simulink model "LQTesting"  (R2025b)
settings: Solver=VariableStepAuto  StartTime=0.0  StopTime=5  RelTol=1e-3
undefined symbols (not defined in the file): ENGINE, IN, K, TANKS, VEH
libraries: simulink_extras x4, aerolibanim x1, matrix_library x1, simulink x1
settings Model: Creator=maxma  LastModifiedBy=maxma

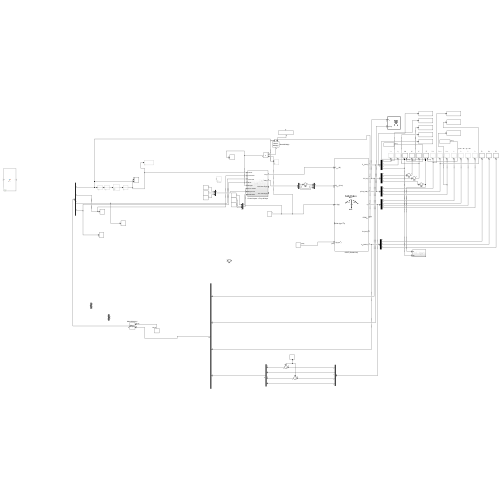
[thumbnail: Simulink's stored preview of the top-level diagram]
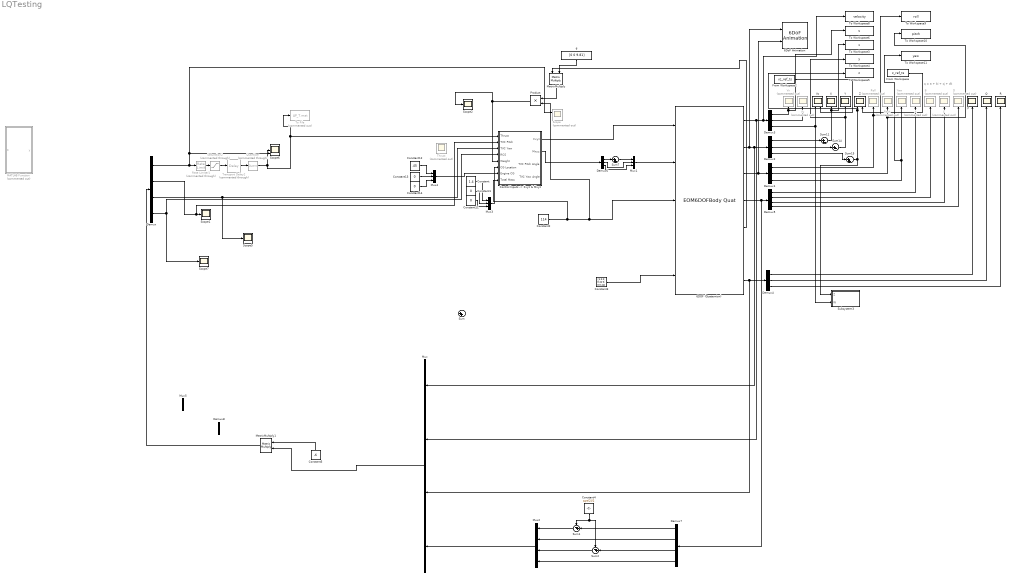
== system LQTesting ==
  note: q = a + bi + cj + dk
  6DOF (Quaternion) : EOM6DOFBodyQuat  mtype=Custom Variable  eul_0=[0 pi/2 0]
  6DoF Animation : aerolibanim/6DoF Animation  u1=[0 200 -200 200 -100 5]  u2=0.1  u3=2  u4=[4000 0 -5000]  u5=Fly alongside  u6=[100 100 -50]  u7=10  u8=on
  A : Scope  Commented=on
      settings: ActiveDisplayYMinimum=-1  ActiveDisplayYMaximum=1  DataLoggingVariableName=ScopeData12
  B : Scope  Commented=on
      settings: ActiveDisplayYMinimum=-1  ActiveDisplayYMaximum=1  DataLoggingVariableName=ScopeData13
  C : Scope  Commented=on
      settings: DataLoggingVariableName=ScopeData14
  Constant : Constant  Value=1.4
  Constant{1,11,13..14} (4 alike) : Constant  Value=0
  Constant12 : Constant  Value=.45
  Constant2 : Constant  Value=114
  Constant3 : Constant  Value=[1 0 0; 0 41 0; 0 0 41]
  Constant4 : Constant  Value=sqrt(2)/2
  Constant5 : Constant  Value=-K
  "Control Inputs -> Fxyz & Mxyz" : Subsystem
  D : Scope  Commented=on
      settings: DataLoggingVariableName=ScopeData15
  Demux{,5,7..8} (4 alike) : Demux
  Demux{1..4,6} (5 alike) : Demux  Outputs=3
  From Workspace : FromWorkspace  VariableName=z_ref_ts
  From Workspace2 : FromWorkspace  VariableName=vz_ref_ts
  MATLAB Function : MATLAB Function  Commented=on  TreatAsAtomicUnit=on
  MatrixMultiply : Product  Multiplication=Matrix(*)
  MatrixMultiply1 : Product  Multiplication=Matrix(*)
  Mux : Mux
  Mux1 : Mux  Inputs=3
  Mux2 : Mux
  Mux3 : Mux  Inputs=3
  Mux4 : Mux  Inputs=3
  Mux5 : Mux  Inputs=2
  P : Scope
      settings: ActiveDisplayYMinimum=-1.1737221275555805  ActiveDisplayYMaximum=1.4340005685452235  DataLoggingVariableName=ScopeData9
  Pitch : Scope  Commented=on
      settings: ActiveDisplayYMinimum=1.5590872483007572  ActiveDisplayYMaximum=1.5720973355164676  DataLoggingVariableName=ScopeData4
  Product : Product
  Q : Scope
      settings: ActiveDisplayYMinimum=-2.1568327186351115  ActiveDisplayYMaximum=1.7945690528650742  DataLoggingVariableName=ScopeData10
  Quantizer : Quantizer  Commented=through  QuantizationInterval=IN.throttle_valve.resolution
  R : Scope
      settings: ActiveDisplayYMinimum=-0.0070860969112896514  ActiveDisplayYMaximum=0.0085398632976064828  DataLoggingVariableName=ScopeData11
  Rate Limiter1 : RateLimiter  Commented=through  RisingSlewLimit=IN.throttle_valve.rate_limit  FallingSlewLimit=-IN.throttle_valve.rate_limit  SampleTimeMode=inherited
  Roll : Scope  Commented=on
      settings: ActiveDisplayYMinimum=-3.9249963147020575  ActiveDisplayYMaximum=3.9253326023284023  DataLoggingVariableName=ScopeData3
  Saturation2 : Saturate  Commented=through  UpperLimit=IN.propulsion.nominal_thrust * IN.propulsion.throttle_range(2)  LowerLimit=IN.propulsion.nominal_thrust * IN.propulsion.throttle_range(1)
  Scope : Scope  Commented=on  NumInputPorts=2
      settings: ActiveDisplayYMinimum=725.64918679567745  ActiveDisplayYMaximum=1423.3753088923004  DataLoggingVariableName=ScopeData52
  Scope{1..2,5,7} (4 alike) : Scope
      Scope1 settings: ActiveDisplayYMinimum=-0.00050229611394169284  ActiveDisplayYMaximum=0.0028458999197228797  DataLoggingVariableName=ScopeData53
      Scope2 settings: DataLoggingVariableName=ScopeData16
      Scope5 settings: ActiveDisplayYMinimum=-16.521850832640737  ActiveDisplayYMaximum=12.974791665814328  DataLoggingVariableName=ScopeData57
      Scope7 settings: ActiveDisplayYMinimum=-140.07362482608556  ActiveDisplayYMaximum=173.20680389636848  DataLoggingVariableName=ScopeData62
  Scope6 : Scope  NumInputPorts=3
      settings: ActiveDisplayYMinimum=-170.62499999999997  ActiveDisplayYMaximum=1535.625  DataLoggingVariableName=ScopeData59
  Subsystem3 : Subsystem
  Sum : Sum  Inputs=|++
  Sum1 : Sum  Inputs=-+|
  Sum11 : Sum  Inputs=|+-
  Sum14 : Sum  Inputs=|+-
  Sum15 : Sum  Inputs=|++
  Sum2 : Sum  Inputs=-+|
  Sum7 : Sum  Inputs=|++
  Thrust : Scope  Commented=on
      settings: ActiveDisplayYMinimum=-220.62499999999994  ActiveDisplayYMaximum=1985.625  DataLoggingVariableName=ScopeData25
  To File : ToFile  Commented=on  Filename=AP_T.mat  SaveFormat=Timeseries
  To Workspace10 : ToWorkspace  VariableName=pitch  SaveFormat=Timeseries  SampleTime=-1
  To Workspace11 : ToWorkspace  VariableName=yaw  SaveFormat=Timeseries  SampleTime=-1
  To Workspace3 : ToWorkspace  VariableName=x  SaveFormat=Timeseries  SampleTime=-1
  To Workspace4 : ToWorkspace  VariableName=y  SaveFormat=Timeseries  SampleTime=-1
  To Workspace5 : ToWorkspace  VariableName=z  SaveFormat=Timeseries  SampleTime=-1
  To Workspace6 : ToWorkspace  VariableName=u  SaveFormat=Timeseries  SampleTime=-1
  To Workspace8 : ToWorkspace  VariableName=velocity  SaveFormat=Timeseries  SampleTime=-1
  To Workspace9 : ToWorkspace  VariableName=roll  SaveFormat=Timeseries  SampleTime=-1
  Transport Delay2 : TransportDelay  Commented=through  DelayTime=IN.throttle_valve_latency
  Vx : Scope  Commented=on
      settings: ActiveDisplayYMinimum=-0.029853358439400533  ActiveDisplayYMaximum=0.01288420382809435  DataLoggingVariableName=ScopeData6
  Vy : Scope  Commented=on
      settings: ActiveDisplayYMinimum=-1  ActiveDisplayYMaximum=1  DataLoggingVariableName=ScopeData7
  Vz : Scope  NumInputPorts=2
      settings: ActiveDisplayYMinimum=-10.206474970594435  ActiveDisplayYMaximum=10.326821590066658  DataLoggingVariableName=ScopeData8
  X : Scope
      settings: ActiveDisplayYMinimum=-0.29732756982374642  ActiveDisplayYMaximum=0.19680411587944552
  Y : Scope
      settings: ActiveDisplayYMinimum=-0.3634591563635699  ActiveDisplayYMaximum=0.16079271216208552
  Yaw : Scope  Commented=on
      settings: ActiveDisplayYMinimum=-0.29772085399940185  ActiveDisplayYMaximum=2.6794861130407197  DataLoggingVariableName=ScopeData5
  Z : Scope  NumInputPorts=2
      settings: ActiveDisplayYMinimum=-86.30767579143982  ActiveDisplayYMaximum=29.689531058480316  DataLoggingVariableName=ScopeData2
  g : Constant  Value=[0 0 9.81]
  wires:
  6DOF (Quaternion)/2 -> 6DoF Animation/1, Mux/1, Demux2/1
  6DOF (Quaternion)/4 -> Demux7/1, Demux5/1
  Demux4/3 -> R/1
  "Control Inputs -> Fxyz & Mxyz"/2(Mxyz) -> Demux6/1
  6DOF (Quaternion)/1 -> Mux/2, To Workspace8/1, Demux3/1
  MatrixMultiply/1 -> Product/1
  Sum14/1 -> To Workspace4/1, Y/1
  Demux6/3 -> Mux1/3
  Demux/4 -> Scope7/1, "Control Inputs -> Fxyz & Mxyz"/4("RCS ")
  Demux5/1 -> A/1
  Demux2/1 -> Sum11/1
  Demux2/3 -> Sum15/1
  Demux5/3 -> C/1
  Demux1/1 -> To Workspace9/1, Roll/1
  Mux1/1 -> 6DOF (Quaternion)/2
  Demux3/1 -> To Workspace6/1, Vx/1
  From Workspace/1 -> Z/2
  Transport Delay2/1 -> Quantizer/1
  Demux4/2 -> Q/1
  Sum15/1 -> Subsystem3/1(Z), To Workspace5/1, Z/1
  g/1 -> MatrixMultiply/2
  Sum11/1 -> To Workspace3/1, X/1
  "Control Inputs -> Fxyz & Mxyz"/1(Fxyz) -> 6DOF (Quaternion)/1
  Saturation2/1 -> Transport Delay2/1
  Quantizer/1 -> "Control Inputs -> Fxyz & Mxyz"/1("Thrust "), To File/1, Scope6/2
  Demux1/2 -> To Workspace10/1, Pitch/1
  Rate Limiter1/1 -> Saturation2/1
  6DOF (Quaternion)/3 -> 6DoF Animation/2, Demux1/1
  Demux/2 -> "Control Inputs -> Fxyz & Mxyz"/2(TVC Pitch), Scope1/1
  Demux3/2 -> Vy/1
  Demux6/1 -> Sum7/1
  Demux4/1 -> P/1
  MatrixMultiply1/1 -> Demux/1
  Demux/1 -> Scope/1, Scope6/3, Rate Limiter1/1
  Demux/3 -> "Control Inputs -> Fxyz & Mxyz"/3(TVC Yaw), Scope5/1
  Demux1/3 -> Yaw/1, To Workspace11/1
  Demux3/3 -> Subsystem3/2(W), Vz/1
  6DOF (Quaternion)/5 -> MatrixMultiply/1
  Demux5/4 -> D/1
  Demux6/2 -> Mux1/2
  Demux2/2 -> Sum14/1
  Sum7/1 -> Mux1/1
  6DOF (Quaternion)/7 -> Mux/3, Demux4/1
  Demux5/2 -> B/1
  From Workspace2/1 -> Vz/2
  Constant2/1 -> Product/2, 6DOF (Quaternion)/3, "Control Inputs -> Fxyz & Mxyz"/8(Total Mass)
  Constant/1 -> Mux3/1
  Constant1/1 -> Mux3/2
  Constant11/1 -> Mux3/3
  Mux3/1 -> "Control Inputs -> Fxyz & Mxyz"/6(CG Location)
  Mux4/1 -> "Control Inputs -> Fxyz & Mxyz"/7(Engine CG)
  Constant12/1 -> Mux4/1
  Constant13/1 -> Mux4/2
  Constant14/1 -> Mux4/3
  Product/1 -> Scope2/1, "Control Inputs -> Fxyz & Mxyz"/5(Weight)
  Constant3/1 -> 6DOF (Quaternion)/5
  Sum1/1 -> Mux2/1
  Mux2/1 -> Mux/4
  Constant4/1 -> Sum1/1, Sum2/1
  Demux7/1 -> Sum1/2
  Demux7/2 -> Mux2/2
  Demux7/3 -> Sum2/2
  Sum2/1 -> Mux2/3
  Demux7/4 -> Mux2/4
  Constant5/1 -> MatrixMultiply1/1
  Mux/1 -> MatrixMultiply1/2

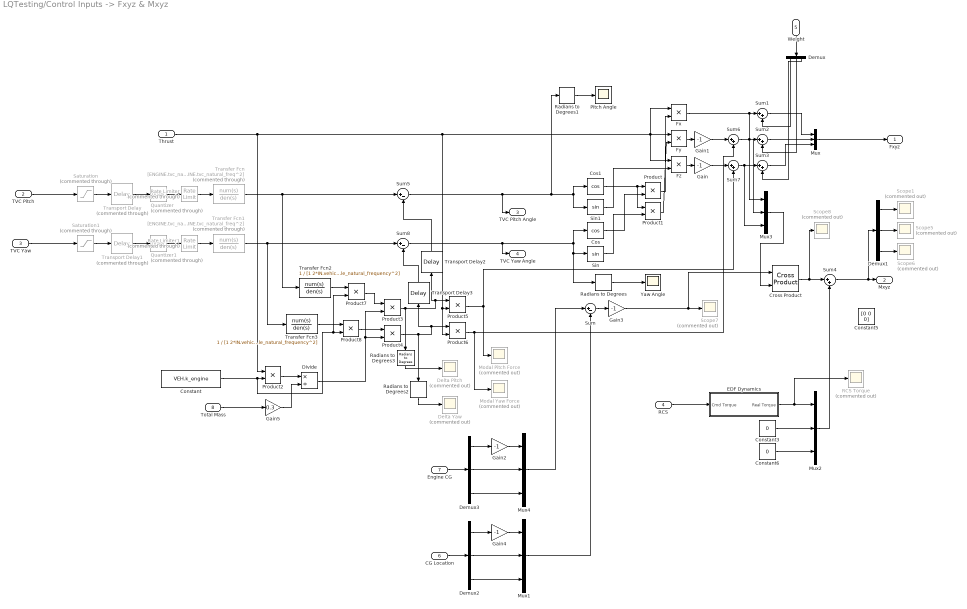
== system LQTesting/Control Inputs -> Fxyz & Mxyz ==
  "Thrust " : Inport
  TVC Pitch : Inport  Port=2
  TVC Yaw : Inport  Port=3
  "RCS " : Inport  Port=4
  Weight : Inport  Port=5
  CG Location : Inport  Port=6
  Engine CG : Inport  Port=7
  Total Mass : Inport  Port=8
  Constant : Constant  Value=VEH.k_engine
  Constant3 : Constant  Value=0
  Constant5 : Constant  Value=[0 0 0]
  Constant6 : Constant  Value=0
  Cos : Trigonometry  Operator=cos
  Cos1 : Trigonometry  Operator=cos
  Cross Product : matrix_library/Cross Product
  Delta Pitch : Scope  Commented=on
      settings: ActiveDisplayYMinimum=-0.004240759901878435  ActiveDisplayYMaximum=0.0031811363034158851  DataLoggingVariableName=ScopeData83
  Delta Yaw : Scope  Commented=on
      settings: ActiveDisplayYMinimum=-0.0055875802598175988  ActiveDisplayYMaximum=0.0072724214879505283  DataLoggingVariableName=ScopeData84
  Demux{,1..3} (4 alike) : Demux  Outputs=3
  Divide : Product  Inputs=*/
  EDF Dynamics : Subsystem
  Fx : Product
  Fy : Product
  Fz : Product
  Gain{,1..4} (5 alike) : Gain  Gain=-1
  Gain5 : Gain  Gain=0.3
  Modal Pitch Force : Scope  Commented=on
      settings: ActiveDisplayYMinimum=-0.0939751193444407  ActiveDisplayYMaximum=0.073347206997115971  DataLoggingVariableName=ScopeData78
  Modal Yaw Force : Scope  Commented=on
      settings: ActiveDisplayYMinimum=-0.12921190722878811  ActiveDisplayYMaximum=0.16063274583799794  DataLoggingVariableName=ScopeData79
  Mux{,1..4} (5 alike) : Mux  Inputs=3
  Pitch Angle : Scope
      settings: ActiveDisplayYMinimum=-1.2449756769959974  ActiveDisplayYMaximum=3.3372562591539077  DataLoggingVariableName=ScopeData71
  Product{,1..8} (9 alike) : Product
  Quantizer : Quantizer  Commented=through  QuantizationInterval=IN.tvc.resolution
  Quantizer1 : Quantizer  Commented=through  QuantizationInterval=IN.tvc.resolution
  RCS Torque : Scope  Commented=on
      settings: ActiveDisplayYMinimum=-11.127953403811379  ActiveDisplayYMaximum=8.61393733576163  DataLoggingVariableName=ScopeData47
  Radians to Degrees{,1..3} (4 alike) : simulink_extras/Transformations/Radians to Degrees
  Rate Limiter : RateLimiter  Commented=through  RisingSlewLimit=IN.tvc.max_gimbal_rate  FallingSlewLimit=-IN.tvc.max_gimbal_rate  SampleTimeMode=inherited
  Rate Limiter1 : RateLimiter  Commented=through  RisingSlewLimit=IN.tvc.max_gimbal_rate  FallingSlewLimit=-IN.tvc.max_gimbal_rate  SampleTimeMode=inherited
  Saturation : Saturate  Commented=through  UpperLimit=IN.tvc.max_gimbal_angle  LowerLimit=-IN.tvc.max_gimbal_angle
  Saturation1 : Saturate  Commented=through  UpperLimit=IN.tvc.max_gimbal_angle  LowerLimit=-IN.tvc.max_gimbal_angle  LinearizeAsGain=off
  Scope{1,5..8} (5 alike) : Scope  Commented=on
      Scope1 settings: ActiveDisplayYMinimum=0.090000000000000011  ActiveDisplayYMaximum=0.11  DataLoggingVariableName=ScopeData50
      Scope5 settings: ActiveDisplayYMinimum=-1  ActiveDisplayYMaximum=1  DataLoggingVariableName=ScopeData54
      Scope6 settings: ActiveDisplayYMinimum=-1  ActiveDisplayYMaximum=1  DataLoggingVariableName=ScopeData55
      Scope7 settings: ActiveDisplayYMinimum=-1.008334185713273  ActiveDisplayYMaximum=-0.924758879501166  DataLoggingVariableName=ScopeData56
      Scope8 settings: ActiveDisplayYMinimum=-1  ActiveDisplayYMaximum=1  DataLoggingVariableName=ScopeData60
  Sin : Trigonometry
  Sin1 : Trigonometry
  Sum : Sum  Inputs=|+-
  Sum{1..4,6..7} (6 alike) : Sum  Inputs=|++
  Sum5 : Sum  Inputs=|+-
  Sum8 : Sum  Inputs=|+-
  Transfer Fcn : TransferFcn  Commented=through  Numerator=[ENGINE.tvc_natural_freq^2]  Denominator=[1 2*IN.tvc.damping_ratio*ENGINE.tvc_natural_freq ENGINE.tvc_natural_freq^2]
  Transfer Fcn1 : TransferFcn  Commented=through  Numerator=[ENGINE.tvc_natural_freq^2]  Denominator=[1 2*IN.tvc.damping_ratio*ENGINE.tvc_natural_freq ENGINE.tvc_natural_freq^2]
  Transfer Fcn2 : TransferFcn  Numerator=1  Denominator=[1 2*IN.vehicle_damping_ratio*IN.vehicle_natural_frequency IN.vehicle_natural_frequency^2]
  Transfer Fcn3 : TransferFcn  Numerator=1  Denominator=[1 2*IN.vehicle_damping_ratio*IN.vehicle_natural_frequency IN.vehicle_natural_frequency^2]
  Transport Delay : TransportDelay  Commented=through  DelayTime=IN.tvc.actuator_latency
  Transport Delay1 : TransportDelay  Commented=through  DelayTime=IN.tvc.actuator_latency
  Transport Delay2 : TransportDelay  DelayTime=0.01
  Transport Delay3 : TransportDelay  DelayTime=0.01
  Yaw Angle : Scope
      settings: ActiveDisplayYMinimum=0.060857666428192986  ActiveDisplayYMaximum=0.32182137924383858  DataLoggingVariableName=ScopeData70
  Fxyz : Outport
  Mxyz : Outport  Port=2
  TVC Pitch Angle : Outport  Port=3
  TVC Yaw Angle : Outport  Port=4
  wires:
  Cos1/1 -> Product1/1, Product/1
  Cos/1 -> Product/2
  Product/1 -> Fx/2
  "Thrust "/1 -> Product2/1, Product6/2, Product5/2, Fx/1, Fy/1, Fz/1
  Mux/1 -> Fxyz/1
  Sum1/1 -> Mux/1
  Weight/1 -> Demux/1
  Fy/1 -> Gain1/1
  Sum2/1 -> Mux/2
  Fz/1 -> Gain/1
  Demux/2 -> Sum2/2
  Mux1/1 -> Sum/2
  Sum/1 -> Gain3/1
  Cross Product/1 -> Scope8/1, Sum4/1
  Constant3/1 -> Mux2/2
  Mux2/1 -> Sum4/2
  Saturation/1 -> Transport Delay/1
  Saturation1/1 -> Transport Delay1/1
  Sum4/1 -> Demux1/1, Mxyz/1
  Demux1/1 -> Scope1/1
  Demux1/2 -> Scope5/1
  Demux1/3 -> Scope6/1
  Product1/1 -> Fy/2
  Sin/1 -> Product1/2
  Sin1/1 -> Fz/2
  Gain3/1 -> Cross Product/1, Scope7/1
  Sum3/1 -> Mux/3
  Mux3/1 -> Cross Product/2
  Constant6/1 -> Mux2/3
  Demux/1 -> Sum1/2
  Demux/3 -> Sum3/2
  Transport Delay/1 -> Quantizer/1
  Transport Delay1/1 -> Quantizer1/1
  Radians to Degrees/1 -> Yaw Angle/1
  Radians to Degrees1/1 -> Pitch Angle/1
  EDF Dynamics/1("Real Torque ") -> RCS Torque/1, Mux2/1
  "RCS "/1 -> EDF Dynamics/1(Cmd Torque)
  Quantizer/1 -> Rate Limiter/1
  Quantizer1/1 -> Rate Limiter1/1
  Rate Limiter/1 -> Transfer Fcn/1
  Rate Limiter1/1 -> Transfer Fcn1/1
  TVC Pitch/1 -> Saturation/1
  TVC Yaw/1 -> Saturation1/1
  Transfer Fcn/1 -> Sum5/1, Transfer Fcn2/1
  Transfer Fcn1/1 -> Sum8/1, Transfer Fcn3/1
  Demux2/3 -> Mux1/3
  CG Location/1 -> Demux2/1
  Demux2/2 -> Mux1/2
  Demux2/1 -> Gain4/1
  Gain4/1 -> Mux1/1
  Gain2/1 -> Mux4/1
  Demux3/1 -> Gain2/1
  Demux3/2 -> Mux4/2
  Demux3/3 -> Mux4/3
  Engine CG/1 -> Demux3/1
  Mux4/1 -> Sum/1
  Total Mass/1 -> Gain5/1
  Product2/1 -> Divide/1
  Gain5/1 -> Divide/2
  Constant/1 -> Product7/2, Product8/2, Product2/2
  Divide/1 -> Product3/2, Product4/2
  Product3/1 -> Transport Delay2/1, Product5/1, Radians to Degrees3/1
  Product4/1 -> Radians to Degrees2/1, Transport Delay3/1, Product6/1
  Fx/1 -> Mux3/1, Sum1/1
  Gain1/1 -> Sum6/1
  Sum6/1 -> Mux3/2, Sum2/1
  Gain/1 -> Sum7/1
  Sum7/1 -> Sum3/1, Mux3/3
  Product5/1 -> Sum7/2, Modal Pitch Force/1
  Product6/1 -> Sum6/2, Modal Yaw Force/1
  Sum5/1 -> TVC Pitch Angle/1, Radians to Degrees1/1, Sin1/1, Cos1/1
  Sum8/1 -> TVC Yaw Angle/1, Sin/1, Radians to Degrees/1, Cos/1
  Radians to Degrees2/1 -> Delta Yaw/1
  Radians to Degrees3/1 -> Delta Pitch/1
  Transport Delay3/1 -> Sum8/2
  Transport Delay2/1 -> Sum5/2
  Transfer Fcn2/1 -> Product7/1
  Product7/1 -> Product3/1
  Transfer Fcn3/1 -> Product8/1
  Product8/1 -> Product4/1

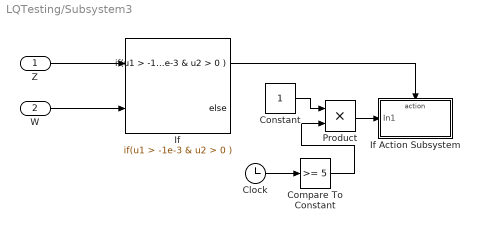
== system LQTesting/Subsystem3 ==
  Z : Inport
  W : Inport  Port=2
  Clock : Clock
  Compare To Constant : simulink/Logic and Bit Operations/Compare To Constant  relop=>=  const=5  OutDataTypeStr=boolean
  Constant : Constant
  If : If  NumInputs=2  IfExpression=u1 > -1e-3 & u2 > 0
  If Action Subsystem : Subsystem  TreatAsAtomicUnit=on
  Product : Product
  wires:
  Z/1 -> If/1
  W/1 -> If/2
  If/1 -> If Action Subsystem/Action
  Clock/1 -> Compare To Constant/1
  Compare To Constant/1 -> Product/2
  Constant/1 -> Product/1
  Product/1 -> If Action Subsystem/1(In1)

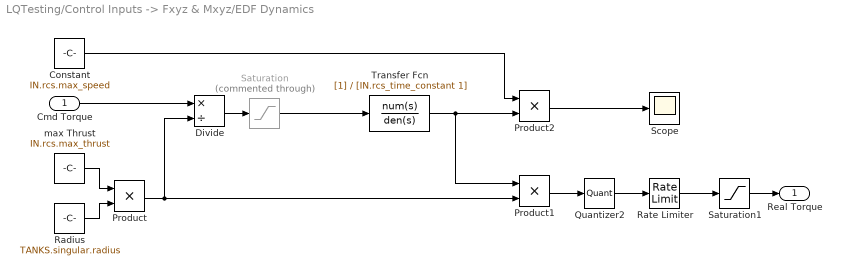
== system LQTesting/Control Inputs -> Fxyz & Mxyz/EDF Dynamics ==
  Cmd Torque : Inport
  Constant : Constant  Value=IN.rcs.max_speed
  Divide : Product  Inputs=*/
  Product : Product
  Product1 : Product
  Product2 : Product
  Quantizer2 : Quantizer  QuantizationInterval=IN.rcs.resolution
  Radius : Constant  Value=TANKS.singular.radius
  Rate Limiter : RateLimiter  RisingSlewLimit=25  FallingSlewLimit=-25  SampleTimeMode=inherited
  Saturation : Saturate  Commented=through  UpperLimit=1  LowerLimit=0  ZeroCross=off
  Saturation1 : Saturate  UpperLimit=IN.rcs.max_thrust  LowerLimit=-IN.rcs.max_thrust  ZeroCross=off
  Scope : Scope
      settings: DataLoggingVariableName=ScopeData48
  Transfer Fcn : TransferFcn  Denominator=[IN.rcs_time_constant 1]
  max Thrust : Constant  Value=IN.rcs.max_thrust
  "Real Torque " : Outport
  wires:
  Constant/1 -> Product2/1
  Divide/1 -> Saturation/1
  Radius/1 -> Product/2
  Product/1 -> Product1/2, Divide/2
  Cmd Torque/1 -> Divide/1
  max Thrust/1 -> Product/1
  Product2/1 -> Scope/1
  Transfer Fcn/1 -> Product2/2, Product1/1
  Product1/1 -> Quantizer2/1
  Saturation/1 -> Transfer Fcn/1
  Quantizer2/1 -> Rate Limiter/1
  Rate Limiter/1 -> Saturation1/1
  Saturation1/1 -> "Real Torque "/1

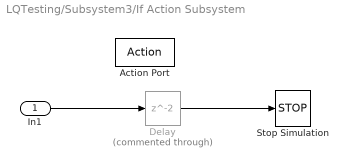
== system LQTesting/Subsystem3/If Action Subsystem ==
  In1 : Inport
  Action Port : ActionPort  ActionPortLabel=|
      | if(u1 > -1e-3 & u2 > 0
      | )
  Delay : Delay  Commented=through
  Stop Simulation : Stop
  wires:
  In1/1 -> Delay/1
  Delay/1 -> Stop Simulation/1

== matlab function LQTesting/MATLAB Function ==
  data: K input; y output
function y = fcn(K)

[A,B,f0] = HopperLinearization_6DOF_LQR(x, u, params)


K =
